simulink model "modulators"  (R2024a)
settings: Solver=VariableStepAuto  StartTime=0.0  StopTime=1  RelTol=1e-3
values from neighbouring files (symbols this model uses):
  fM = fM_vector(j)    [tradeoff.m]
undefined symbols (not defined in the file or in its folder): DiscIntNeverNeededParam
libraries: simulink_extras x6
settings Model: Creator=rjtg2  LastModifiedBy=rjtg2

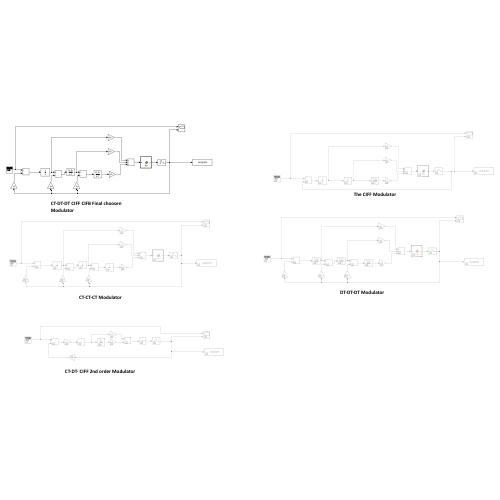
[thumbnail: Simulink's stored preview of the top-level diagram]
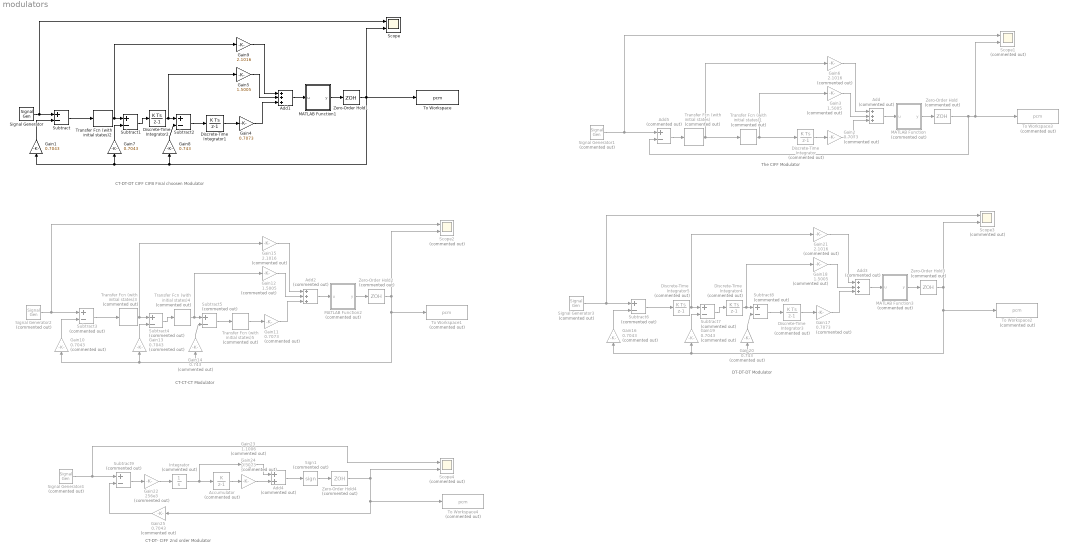
== system modulators ==
  note: The CIFF Modulator
  note: CT-DT-DT CIFF CIFB Final choosen Modulator
  note: CT-CT-CT Modulator
  note: DT-DT-DT Modulator
  note: CT-DT- CIFF 2nd order Modulator
  Accumulator : DiscreteIntegrator  Commented=on  IntegratorMethod=Accumulation: Forward Euler  SampleTime=1/fM  ICPrevOutput=DiscIntNeverNeededParam  ICPrevScaledInput=DiscIntNeverNeededParam
  Add : Sum  Commented=on  Inputs=+++
  Add1 : Sum  Inputs=+++
  Add2 : Sum  Commented=on  Inputs=+++
  Add3 : Sum  Commented=on  Inputs=+++
  Add4 : Sum  Commented=on
  Add5 : Sum  Commented=on  Inputs=+-
  Discrete-Time Integrator{,3..5} (4 alike) : DiscreteIntegrator  Commented=on  gainval=1  SampleTime=1/fM  UpperSaturationLimit=+2  LowerSaturationLimit=-2  ICPrevOutput=DiscIntNeverNeededParam  ICPrevScaledInput=DiscIntNeverNeededParam
  Discrete-Time Integrator1 : DiscreteIntegrator  gainval=1  SampleTime=1/fM  UpperSaturationLimit=+2  LowerSaturationLimit=-2  ICPrevOutput=DiscIntNeverNeededParam  ICPrevScaledInput=DiscIntNeverNeededParam
  Discrete-Time Integrator2 : DiscreteIntegrator  gainval=1  SampleTime=1/fM  UpperSaturationLimit=+2  LowerSaturationLimit=-2  ICPrevOutput=DiscIntNeverNeededParam  ICPrevScaledInput=DiscIntNeverNeededParam
  Gain1 : Gain  Gain=0.7043
  Gain{10,13,16,19,25} (5 alike) : Gain  Commented=on  Gain=0.7043
  Gain11 : Gain  Commented=on  Gain=0.7073
  Gain12 : Gain  Commented=on  Gain=1.5005
  Gain14 : Gain  Commented=on  Gain=0.743
  Gain15 : Gain  Commented=on  Gain=2.1016
  Gain17 : Gain  Commented=on  Gain=0.7073
  Gain18 : Gain  Commented=on  Gain=1.5005
  Gain2 : Gain  Commented=on  Gain=0.7073
  Gain20 : Gain  Commented=on  Gain=0.743
  Gain21 : Gain  Commented=on  Gain=2.1016
  Gain22 : Gain  Commented=on  Gain=256e3
  Gain23 : Gain  Commented=on  Gain=1.1006
  Gain24 : Gain  Commented=on  Gain=0.3073
  Gain3 : Gain  Commented=on  Gain=1.5005
  Gain4 : Gain  Gain=0.7073
  Gain5 : Gain  Gain=1.5005
  Gain6 : Gain  Commented=on  Gain=2.1016
  Gain7 : Gain  Gain=0.7043
  Gain8 : Gain  Gain=0.743
  Gain9 : Gain  Gain=2.1016
  Integrator : Integrator  Commented=on
  MATLAB Function : MATLAB Function  Commented=on  TreatAsAtomicUnit=on
  MATLAB Function1 : MATLAB Function  TreatAsAtomicUnit=on
  MATLAB Function2 : MATLAB Function  Commented=on  TreatAsAtomicUnit=on
  MATLAB Function3 : MATLAB Function  Commented=on  TreatAsAtomicUnit=on
  Scope : Scope  NumInputPorts=2
  Scope{1..4} (4 alike) : Scope  Commented=on  NumInputPorts=2
  Sign1 : Signum  Commented=on
  Signal Generator : SignalGenerator  Frequency=1000
  Signal Generator1 : SignalGenerator  Commented=on  Frequency=1000
  Signal Generator2 : SignalGenerator  Commented=on  Frequency=1000
  Signal Generator3 : SignalGenerator  Commented=on  Frequency=1000
  Signal Generator4 : SignalGenerator  Commented=on  Amplitude=0.5  Frequency=1000
  Subtract : Sum  Inputs=+-
  Subtract1 : Sum  Inputs=+-
  Subtract2 : Sum  Inputs=+-
  Subtract{3..9} (7 alike) : Sum  Commented=on  Inputs=+-
  To Workspace : ToWorkspace  VariableName=pcm  SaveFormat=Timeseries  SampleTime=-1
  To Workspace{1..4} (4 alike) : ToWorkspace  Commented=on  VariableName=pcm  SampleTime=-1
  Transfer Fcn (with initial states){,1,3..5} (5 alike) : simulink_extras/Additional Linear/Transfer Fcn (with initial states)  Commented=on  N=[1]  D=[1 0]  X0=0
  Transfer Fcn (with initial states)2 : simulink_extras/Additional Linear/Transfer Fcn (with initial states)  N=[1]  D=[1 0]  X0=0
  Zero-Order Hold{,2..4} (4 alike) : ZeroOrderHold  Commented=on  SampleTime=1/fM
  Zero-Order Hold1 : ZeroOrderHold  SampleTime=1/fM
  wires:
  Transfer Fcn (with initial states)1/1 -> Discrete-Time Integrator/1, Gain3/1
  Signal Generator1/1 -> Add5/1, Scope1/1
  Gain2/1 -> Add/3
  Discrete-Time Integrator/1 -> Gain2/1
  MATLAB Function/1(y) -> Zero-Order Hold/1
  Transfer Fcn (with initial states)/1 -> Transfer Fcn (with initial states)1/1, Gain6/1
  Zero-Order Hold/1 -> Add5/2, To Workspace3/1, Scope1/2
  Add/1 -> MATLAB Function/1(u)
  Gain3/1 -> Add/2
  Gain6/1 -> Add/1
  Signal Generator/1 -> Scope/1, Subtract/1
  Gain4/1 -> Add1/3
  Discrete-Time Integrator2/1 -> Gain5/1, Subtract2/1
  Discrete-Time Integrator1/1 -> Gain4/1
  Gain8/1 -> Subtract2/2
  Subtract2/1 -> Discrete-Time Integrator1/1
  Subtract/1 -> Transfer Fcn (with initial states)2/1
  Gain1/1 -> Subtract/2
  Add1/1 -> MATLAB Function1/1(u)
  Subtract1/1 -> Discrete-Time Integrator2/1
  Transfer Fcn (with initial states)2/1 -> Subtract1/1, Gain9/1
  Gain5/1 -> Add1/2
  MATLAB Function1/1(y) -> Zero-Order Hold1/1
  Zero-Order Hold1/1 -> To Workspace/1, Scope/2, Gain8/1, Gain7/1, Gain1/1
  Gain7/1 -> Subtract1/2
  Gain9/1 -> Add1/1
  Gain11/1 -> Add2/3
  Gain12/1 -> Add2/2
  Zero-Order Hold2/1 -> Scope2/2, Gain14/1, Gain13/1, Gain10/1, To Workspace1/1
  Add2/1 -> MATLAB Function2/1(u)
  Gain14/1 -> Subtract5/2
  Gain13/1 -> Subtract4/2
  Transfer Fcn (with initial states)3/1 -> Subtract4/1, Gain15/1
  Gain15/1 -> Add2/1
  Subtract5/1 -> Transfer Fcn (with initial states)5/1
  Subtract3/1 -> Transfer Fcn (with initial states)3/1
  Transfer Fcn (with initial states)4/1 -> Gain12/1, Subtract5/1
  Transfer Fcn (with initial states)5/1 -> Gain11/1
  MATLAB Function2/1(y) -> Zero-Order Hold2/1
  Gain10/1 -> Subtract3/2
  Signal Generator2/1 -> Scope2/1, Subtract3/1
  Subtract4/1 -> Transfer Fcn (with initial states)4/1
  Gain19/1 -> Subtract7/2
  Discrete-Time Integrator3/1 -> Gain17/1
  Subtract8/1 -> Discrete-Time Integrator3/1
  Subtract6/1 -> Discrete-Time Integrator5/1
  MATLAB Function3/1(y) -> Zero-Order Hold3/1
  Gain17/1 -> Add3/3
  Gain21/1 -> Add3/1
  Zero-Order Hold3/1 -> Scope3/2, To Workspace2/1, Gain20/1, Gain19/1, Gain16/1
  Add3/1 -> MATLAB Function3/1(u)
  Gain20/1 -> Subtract8/2
  Discrete-Time Integrator4/1 -> Gain18/1, Subtract8/1
  Gain16/1 -> Subtract6/2
  Gain18/1 -> Add3/2
  Subtract7/1 -> Discrete-Time Integrator4/1
  Discrete-Time Integrator5/1 -> Subtract7/1, Gain21/1
  Signal Generator3/1 -> Scope3/1, Subtract6/1
  Gain22/1 -> Integrator/1
  Zero-Order Hold4/1 -> Scope4/2, To Workspace4/1, Gain25/1
  Gain23/1 -> Add4/1
  Accumulator/1 -> Gain24/1
  Add4/1 -> Sign1/1
  Signal Generator4/1 -> Scope4/1, Subtract9/1
  Gain25/1 -> Subtract9/2
  Gain24/1 -> Add4/2
  Sign1/1 -> Zero-Order Hold4/1
  Integrator/1 -> Accumulator/1, Gain23/1
  Subtract9/1 -> Gain22/1
  Add5/1 -> Transfer Fcn (with initial states)/1

== matlab function modulators/MATLAB Function ==
  data: u input; y output
function y = fcn(u)
    if u >= 0
        y = 1;
    else 
        y = -1;
    end

== matlab function modulators/MATLAB Function2 ==
  data: u input; y output
function y = fcn(u)
    if u >= 0
        y = 1;
    else 
        y = -1;
    end

== matlab function modulators/MATLAB Function3 ==
  data: u input; y output
function y = fcn(u)
    if u >= 0
        y = 1.8;
    else 
        y = -1.8;
    end

== matlab function modulators/MATLAB Function1 ==
  data: u input; y output
function y = fcn(u)
    if u >= 0
        y = 1;
    else 
        y = -1;
    end
